simulink model "bldcControl"  (R2021b)
settings: Solver=VariableStepAuto  StartTime=0.0  StopTime=0.3  RelTol=1e-3
InitFcn:
  | modelData;
undefined symbols (not defined in the file or in its folder): inverter, motor
libraries: simulink x26, nesl_utility x13, fl_lib x7, ee_lib x6, simulink_extras x1
settings Model: Creator=andre  LastModifiedBy=andre
settings SolverCC: AlgebraicLoopSolver=TrustRegion
settings DebuggingCC: SFMachineParentedDataDiag=warning

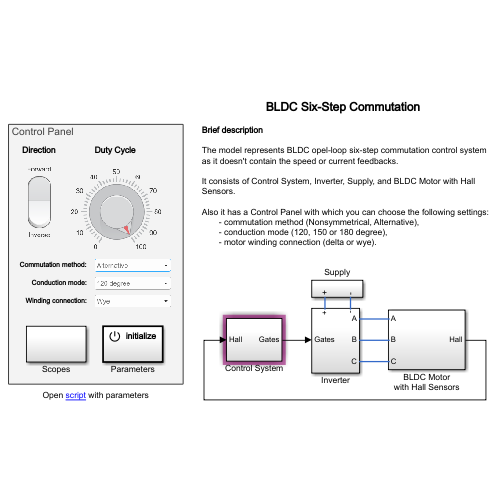
[thumbnail: Simulink's stored preview of the top-level diagram]
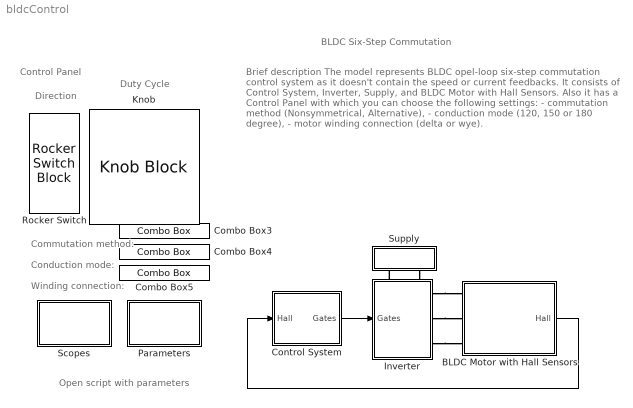
== system bldcControl ==
  note: Brief description
      |
      | The model represents BLDC opel-loop six-step commutation control system as it doesn't contain the speed or current feedbacks.
      |
      | It consists of Control System, Inverter, Supply, and BLDC Motor with Hall Sensors.
      |
      | Also it has a Control Panel with which you can choose the following settings: - commutation method (Nonsymmetrical, Alternative),
      | - conduction mode (120, 150 or 180 degree),
      | - motor winding connection (delta or wye).
  note: BLDC Six-Step Commutation
  note: Open script with parameters
  note: Direction
  note: Duty Cycle
  note: Commutation method:
  note: Control Panel
  note: Conduction mode:
  note: Winding connection:
  BLDC Motor with Hall Sensors : Subsystem
  Combo Box3 : ComboBox  LabelPosition=Hide  SelectedLabel=Alternative
      settings: Values={{'Nonsymmetrical (down)', 'Nonsymmetrical (up)', 'Alternative'}, [0 100 50]}
  Combo Box4 : ComboBox  LabelPosition=Hide  SelectedLabel=120 degree
      settings: Values={{'120 degree', '150 degree', '180 degree'}, [1 2 3]}
  Combo Box5 : ComboBox  LabelPosition=Hide  SelectedLabel=Wye
      settings: Values={{'Delta', 'Wye'}, [1 2]}
  Control System : Subsystem
  Inverter : Subsystem
      settings: PortSchema="{\"entries\":[{\"content\":{\"sides\":[{\"content\":{\"connectorIds\":[\"In1\"]},\"type\":\"ConnectorPlacement.EquallySpacedRectSide\",\"uuid\":\"39f629fa-0bd2-4f88-acf3-917ef1f8012c\"},{\"content\":{\"connectorIds\":[\"RConn1\",\"RConn2\",\"RConn3\"],\"side\":\"RIGHT\"},\"type\":\"ConnectorPlacement.EquallySpacedRectSide\",\"uuid\":\"8e31936c-1fbb-4376-88bf-295b0c5638c2\"},{\"content\":{\"connectorIds\":[\"LConn1\",\"LConn2\"],\"side\":\"TOP\"},\"type\":\"ConnectorPlacement.EquallySpacedRectSide\",\"uuid\":\"2e7c4c30-56fe-4abf-adf0-7801e76feedc\"},{\"content\":{\"connectorIds\":[],\"side\":\"BOTTOM\"},\"type\":\"ConnectorPlacement.EquallySpacedRectSide\",\"uuid\":\"fe44a21b-96bc-40f6-9ec6-e237835ad4c0\"},{\"content\":{\"connectorIds\":[],\"side\":\"HIDDEN\"},\"type\":\"ConnectorPlacement.EquallySpacedRectSide\",\"uuid\":\"0ee61edf-83e7-441c-a702-98ac80ee1211\"}]},\"type\":\"ConnectorPlacement.EquallySpacedConnector\",\"uuid\":\"7a564375-3113-4624-a173-7e6d668cb20c\"}],\"packageUris\":[\"http://schema.mathworks.com/mf0/Connector/R2020b\"],\"version\":\"1.0\"}"
  Knob : KnobBlock  LabelPosition=Hide  TickInterval=10
  Parameters : Subsystem  TreatAsAtomicUnit=on
  Rocker Switch : RockerSwitchBlock  LabelPosition=Hide
      settings: Values={{'Inverse', 'Forward'}, [1 0]}
  Scopes : Subsystem
  Supply : Subsystem
  wires:
  Control System/1(Gates) -> Inverter/1(Gates)
  BLDC Motor with Hall Sensors/1(Hall) -> Control System/1(Hall)
  connections:
  Inverter/RConn1 -- BLDC Motor with Hall Sensors/LConn1
  Supply/RConn2 -- Inverter/LConn2
  Inverter/RConn3 -- BLDC Motor with Hall Sensors/LConn3
  Inverter/RConn2 -- BLDC Motor with Hall Sensors/LConn2
  Inverter/LConn1 -- Supply/RConn1

== system bldcControl/BLDC Motor with Hall Sensors ==
  Hall Sensors : Subsystem
  Mechanical Rotational Reference1 : fl_lib/Mechanical/Rotational Elements/Mechanical Rotational Reference
  Motor : Subsystem  Variant=on
  A : PMIOPort  Side=Left
  B : PMIOPort  Port=2  Side=Left
  C : PMIOPort  Port=3  Side=Left
  Hall : Outport
  wires:
  Hall Sensors/1(Hall) -> Hall/1
  connections:
  Motor/LConn1 -- A/RConn1
  Motor/RConn1 -- Hall Sensors/LConn1
  Motor/LConn3 -- C/RConn1
  Motor/LConn2 -- B/RConn1
  Mechanical Rotational Reference1/LConn1 -- Motor/RConn2

== system bldcControl/Control System ==
  note: The control system is based on six-step commutation technique
      | which uses 120-degree, 150-degree, and 180-degree conduction modes.
      |
      | This control is described with the thuth table of 5 logical variables:
      | 1. DR (DiRection) is direction of the motor rotation
      | (0 - forward direction, 1 - inverse direction);
      | 2. H - Hall sensors signals;
      | 3. PR (PRoportion) determines the loading of switches
      | (PWM-based variable);
      | 4. SP (SPeed) is relative speed (PWM-based variable).
      |
      | When CM = 0, PR = 0 and lower switches are loaded more than
      | upper ones. When CM = 100, PR = 1 and upper switches are loaded
      | more than lower ones. When CM = 50, PR = 0.5, it means that
      | upper and lower switched are loaded uniformly during the commutation
      | interval.
      |
      | The commutation modes are called nonsymmentrical (down),
      | nonsymmentrical (up), and alternative, respectively.
  note: Description of commutation technique
  Hall : Inport
  CM : Constant  Value=50
  Direction : Constant  Value=0
  Duty Cycle : Constant  Value=100
  Logical variables formation : Subsystem
  Truth Tables : Subsystem  Variant=on
  Gates : Outport
  tag scope: Gates=global
  wires:
  Direction/1 -> Logical variables formation/1(DR)
  Hall/1 -> Logical variables formation/2(H)
  CM/1 -> Logical variables formation/3(PR)
  Duty Cycle/1 -> Logical variables formation/4(SP)
  Logical variables formation/1(LV) -> Truth Tables/1(LV)
  Truth Tables/1(Gates) -> Gates/1, [Gates]

== system bldcControl/Inverter ==
  Gates : Inport
  Converter (Three-Phase) : ee_lib/Semiconductors & Converters/Converters/Converter (Three-Phase)  port_option=ee.enum.threePhasePort.expanded  device_type=ee.enum.converters.switchingdevice.mosfet  Vf=0.8 V  Ron=4e-2 Ohm  Rds=inverter.Rds Ohm  Goff=inverter.Goffs 1/Ohm  Vgt=1 V  Vgt_off=-1 V  Ih=1 A  Vth=inverter.Uthr V  diode_param=ee.enum.converters.protectiondiode.nodynamics  diode_Vf=inverter.Udf V  diode_Ron=inverter.Ron Ohm  diode_Goff=inverter.Goff 1/Ohm  diode_C=50 nF  diode_iRM=-235 A  diode_iF=300 A  diode_idot=-50 A/us  diode_trr_param=ee.enum.converters.diodetrr.trr_factor  diode_trr_factor=3  diode_trr=15 us  diode_Qrr=1500 s*uA  snubber_type=ee.enum.converters.snubber.include  Cs=inverter.Csn F  Rs="inverter.Rsn  Ohm"
      settings: SourceProductBaseCode=PS  InternalSimscapePortConfiguration="{\"Bottom\":[],\"Left\":[{\"id\":\"G\",\"label\":\"G\",\"type\":\"foundation.electrical.twelve_phase\"},{\"id\":\"a\",\"label\":\"a\",\"type\":\"foundation.electrical.electrical\"},{\"id\":\"b\",\"label\":\"b\",\"type\":\"foundation.electrical.electrical\"},{\"id\":\"c\",\"label\":\"c\",\"type\":\"foundation.electrical.electrical\"}],\"Right\":[{\"id\":\"p\",\"label\":\"+\",\"type\":\"foundation.electrical.electrical\"},{\"id\":\"n\",\"label\":\"-\",\"type\":\"foundation.electrical.electrical\"}],\"Top\":[]}"
  Gate Driver : Subsystem
  Subsystem : Subsystem
      mask Display: disp('M')
  + : PMIOPort  Side=Left
  - : PMIOPort  Port=2  Side=Left
  A : PMIOPort  Port=3  Side=Right
  B : PMIOPort  Port=4  Side=Right
  C : PMIOPort  Port=5  Side=Right
  wires:
  Gates/1 -> Gate Driver/1(S)
  connections:
  Gate Driver/RConn1 -- Converter (Three-Phase)/LConn1
  Subsystem/RConn2 -- B/RConn1
  +/RConn1 -- Converter (Three-Phase)/RConn1
  Subsystem/LConn2 -- Converter (Three-Phase)/LConn3
  Subsystem/LConn3 -- Converter (Three-Phase)/LConn4
  Subsystem/LConn1 -- Converter (Three-Phase)/LConn2
  -/RConn1 -- Converter (Three-Phase)/RConn2
  Subsystem/RConn1 -- A/RConn1
  Subsystem/RConn3 -- C/RConn1

== system bldcControl/Parameters ==
  Control method : Constant
  Event Listener : EventListener  DisableCoverage=on  EventName=reset
  Terminator : Terminator
  Terminator1 : Terminator
  Wound type : Constant  Value=2
  wires:
  Control method/1 -> Terminator/1
  Wound type/1 -> Terminator1/1

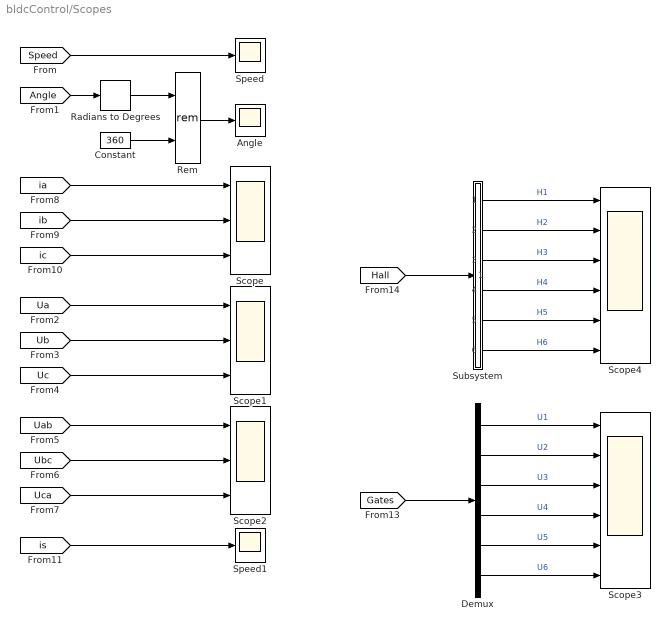
== system bldcControl/Scopes ==
  Angle : Scope
  Constant : Constant  Value=360
  Demux : Demux  Outputs=6
  Radians to Degrees : simulink_extras/Transformations/Radians to Degrees
  Rem : Math  Operator=rem  SaturateOnIntegerOverflow=on
  Scope : Scope  NumInputPorts=3
  Scope1 : Scope  NumInputPorts=3
  Scope2 : Scope  NumInputPorts=3
  Scope3 : Scope  NumInputPorts=6
  Scope4 : Scope  NumInputPorts=6
  Speed : Scope
  Speed1 : Scope
  Subsystem : Subsystem
  wires:
  [Angle] -> Radians to Degrees/1
  [ib] -> Scope/2
  [ia] -> Scope/1
  [ic] -> Scope/3
  [Ub] -> Scope1/2
  [Ua] -> Scope1/1
  [Uc] -> Scope1/3
  [Ubc] -> Scope2/2
  [Uab] -> Scope2/1
  [Uca] -> Scope2/3
  Rem/1 -> Angle/1
  Radians to Degrees/1 -> Rem/1
  Constant/1 -> Rem/2
  [is] -> Speed1/1
  [Speed] -> Speed/1
  [Gates] -> Demux/1
  [Hall] -> Subsystem/1(In1)
  Demux/1 -> Scope3/1  "U1"
  Demux/2 -> Scope3/2  "U2"
  Demux/3 -> Scope3/3  "U3"
  Demux/4 -> Scope3/4  "U4"
  Demux/5 -> Scope3/5  "U5"
  Demux/6 -> Scope3/6  "U6"
  Subsystem/1(H1) -> Scope4/1  "H1"
  Subsystem/2(H2) -> Scope4/2  "H2"
  Subsystem/3(H3) -> Scope4/3  "H3"
  Subsystem/4(H4) -> Scope4/4  "H4"
  Subsystem/5(H5) -> Scope4/5  "H5"
  Subsystem/6(H6) -> Scope4/6  "H6"

== system bldcControl/Supply ==
  DC Voltage Source : fl_lib/Electrical/Electrical Sources/DC Voltage Source  v0=motor.Us V
  Electrical Reference2 : fl_lib/Electrical/Electrical Elements/Electrical Reference
  Solver Configuration : nesl_utility/Solver Configuration  PhysicalDomain=network_engine_domain  SubClassName=solver  LeftPortType=input  RightPortType=generic  Tones=[]  Harmonics=[]  SimulateNoise=off  Profile=off  UseLocalSampling=off  EnableSwitchedLinearOptims=on  FrequencyDomain=off  UseCCode=off  RelTol=0.001  AbsTol=1e-06  MinStep=1e-09  ToWorkspace=off  RevertToSquareIcSolve=off  NumHomotopyIterations=100  PhasorMode=off  PhasorModeNumHarmonics=1  DoDC=off  ResidualTolerance=1e-09  UseLocalSolver=on  LocalSolverChoice=NE_BACKWARD_EULER_ADVANCER  LocalSolverSampleTime=Ts  DoFixedCost=on  MaxNonlinIter=4  MaxModeIter=2  ComputeImpulses=off  ImpulseIterations=2  LinearAlgebra=auto  EquationFormulation=NE_TIME_EF  DelaysMemoryBudget=1024  AutomaticFiltering=off  FilteringTimeConstant=0.001  PartitionStorageMethod=AS_NEEDED  PartitionMemoryBudget=1024  PartitionMethod=ROBUST
      settings: SourceProductBaseCode=PW,SS
  Subsystem : Subsystem
      mask Display: disp('A')
  + : PMIOPort  Side=Right
  - : PMIOPort  Port=2  Side=Right
  connections:
  DC Voltage Source/RConn1 -- Electrical Reference2/LConn1 -- Solver Configuration/RConn1 -- -/RConn1
  Subsystem/RConn1 -- +/RConn1
  Subsystem/LConn1 -- DC Voltage Source/LConn1

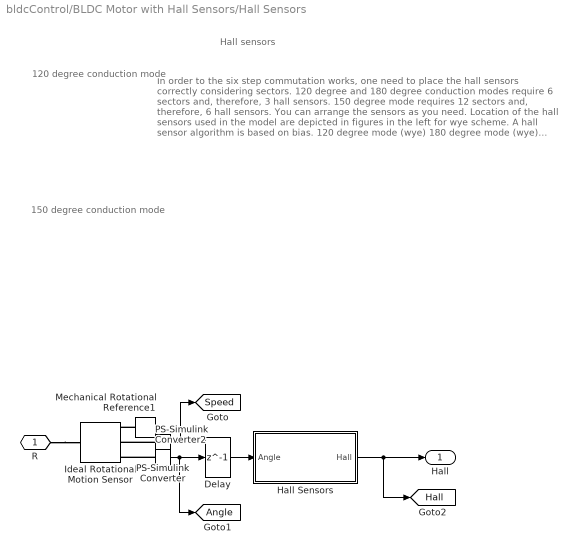
== system bldcControl/BLDC Motor with Hall Sensors/Hall Sensors ==
  note: In order to the six step commutation works, one need to place the hall sensors correctly considering sectors.
      |
      | 120 degree and 180 degree conduction modes require 6 sectors and, therefore, 3 hall sensors. 150 degree mode requires 12 sectors and, therefore, 6 hall sensors.
      |
      | You can arrange the sensors as you need. Location of the hall sensors used in the model are depicted in figures in the left for wye scheme.
      |
      | A hall sensor algorithm is based on bias.
      |
      | 120 degree mode (wye)    180 degree mode (wye)    150 degree mode (wye)
      | 	H   | Bias				H   | Bias				H   | Bias
      | 	H1 | 0					H1 | -pi/6				H1 | pi/3
      | 	H2 | 2*pi/3				H2 | pi/2					H2 | pi/6
      | 	H3 | -2*pi/3				H3 | -5*pi/6				H3 | 0
      | 													H4 | -pi/6
      | 													H5 | -pi/3
      | 													H6 | -pi/2
      |
      | For delta scheme, all corresponding hall sensors are moved clockwise
      | by 30 degrees relative to wye scheme.
  note: 120 degree
      | conduction mode
  note: Hall sensors
  note: 150 degree
      | conduction mode
  Delay : Delay  DelayLength=1
  Hall Sensors : Subsystem  Variant=on
  Ideal Rotational Motion Sensor : fl_lib/Mechanical/Mechanical Sensors/Ideal Rotational Motion Sensor  wrap_angle=simscape.enum.onoff.off  offset=0 deg
  Mechanical Rotational Reference1 : fl_lib/Mechanical/Rotational Elements/Mechanical Rotational Reference
  PS-Simulink Converter : nesl_utility/PS-Simulink Converter  PhysicalDomain=network_engine_domain  SubClassName=ps_output  LeftPortType=input  RightPortType=output  PseudoPeriodic=off  Frequencies=[]  Unit=rpm  AffineConversion=off
      settings: SourceProductBaseCode=PW,SS
  PS-Simulink Converter2 : nesl_utility/PS-Simulink Converter  PhysicalDomain=network_engine_domain  SubClassName=ps_output  LeftPortType=input  RightPortType=output  PseudoPeriodic=off  Frequencies=[]  Unit=rad  AffineConversion=off
      settings: SourceProductBaseCode=PW,SS
  R : PMIOPort  Side=Left
  Hall : Outport
  tag scope: Angle=global, Hall=global, Speed=global
  wires:
  Delay/1 -> Hall Sensors/1(Angle)
  PS-Simulink Converter2/1 -> [Angle], Delay/1
  Hall Sensors/1(Hall) -> [Hall], Hall/1
  PS-Simulink Converter/1 -> [Speed]
  connections:
  PS-Simulink Converter2/LConn1 -- Ideal Rotational Motion Sensor/RConn3
  PS-Simulink Converter/LConn1 -- Ideal Rotational Motion Sensor/RConn2
  Mechanical Rotational Reference1/LConn1 -- Ideal Rotational Motion Sensor/RConn1
  R/RConn1 -- Ideal Rotational Motion Sensor/LConn1

== system bldcControl/BLDC Motor with Hall Sensors/Motor ==
  Delta : Subsystem  VariantControl=DELTA_WOUND
  Wye : Subsystem  VariantControl=WYE_WOUND
  A : PMIOPort  Side=Left
  B : PMIOPort  Port=2  Side=Left
  C : PMIOPort  Port=3  Side=Left
  R : PMIOPort  Port=4  Side=Right
  Сase : PMIOPort  Port=5  Side=Right

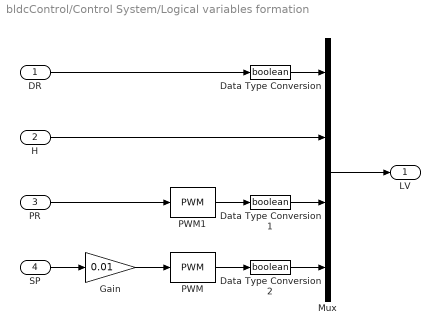
== system bldcControl/Control System/Logical variables formation ==
  DR : Inport
  H : Inport  Port=2
  PR : Inport  Port=3
  SP : Inport  Port=4
  Data Type Conversion : DataTypeConversion  OutDataTypeStr=boolean
  Data Type Conversion1 : DataTypeConversion  OutDataTypeStr=boolean
  Data Type Conversion2 : DataTypeConversion  OutDataTypeStr=boolean
  Gain : Gain  Gain=0.01
  Mux : Mux
  PWM : simulink/Discontinuities/PWM  DisableCoverage=on  Period=1/inverter.f  DisallowZeroDutyCycle=off  RunAtFixedTimeIntervals=off  SampleTime=0.1
  PWM1 : simulink/Discontinuities/PWM  DisableCoverage=on  Period=2/inverter.f  DisallowZeroDutyCycle=off  RunAtFixedTimeIntervals=off  SampleTime=0.1
  LV : Outport
  wires:
  Data Type Conversion/1 -> Mux/1
  DR/1 -> Data Type Conversion/1
  SP/1 -> Gain/1
  PR/1 -> PWM1/1
  PWM1/1 -> Data Type Conversion1/1
  Gain/1 -> PWM/1
  PWM/1 -> Data Type Conversion2/1
  Data Type Conversion1/1 -> Mux/3
  Mux/1 -> LV/1
  Data Type Conversion2/1 -> Mux/4
  H/1 -> Mux/2

== system bldcControl/Control System/Truth Tables ==
  LV : Inport
  120 degree : Subsystem  VariantControl=DEG120
  150 degree : Subsystem  VariantControl=DEG150
  180 degree : Subsystem  VariantControl=DEG180
  Gates : Outport

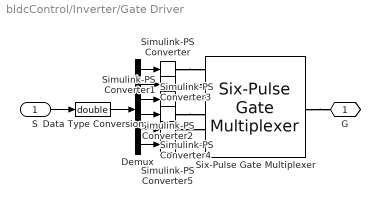
== system bldcControl/Inverter/Gate Driver ==
  S : Inport
  Data Type Conversion : DataTypeConversion  OutDataTypeStr=double
  Demux : Demux  Outputs=6
  Simulink-PS Converter{,1..5} (6 alike) : nesl_utility/Simulink-PS Converter  PhysicalDomain=network_engine_domain  SubClassName=ps_input  LeftPortType=input  RightPortType=output  PseudoPeriodic=off  Frequencies=[]  NoiseDistribution=none  NoiseParameters=[]  Unit=1  AffineConversion=off  FilteringAndDerivatives=provide  SimscapeFilterOrder=1  InputFilterTimeConstant=0.001  UdotUserProvided=0
      settings: SourceProductBaseCode=PW,SS
  Six-Pulse Gate Multiplexer : ee_lib/Semiconductors & Converters/Converters/Six-Pulse Gate Multiplexer  port_option=ee.enum.controlport.ps
      settings: SourceProductBaseCode=PS
  G : PMIOPort  Side=Right
  wires:
  Demux/3 -> Simulink-PS Converter2/1
  Demux/2 -> Simulink-PS Converter1/1
  Demux/6 -> Simulink-PS Converter5/1
  Demux/5 -> Simulink-PS Converter4/1
  Demux/4 -> Simulink-PS Converter3/1
  Demux/1 -> Simulink-PS Converter/1
  Data Type Conversion/1 -> Demux/1
  S/1 -> Data Type Conversion/1
  connections:
  Simulink-PS Converter4/RConn1 -- Six-Pulse Gate Multiplexer/LConn5
  Six-Pulse Gate Multiplexer/LConn6 -- Simulink-PS Converter5/RConn1
  Simulink-PS Converter3/RConn1 -- Six-Pulse Gate Multiplexer/LConn4
  Simulink-PS Converter1/RConn1 -- Six-Pulse Gate Multiplexer/LConn2
  Six-Pulse Gate Multiplexer/LConn3 -- Simulink-PS Converter2/RConn1
  Simulink-PS Converter/RConn1 -- Six-Pulse Gate Multiplexer/LConn1
  Six-Pulse Gate Multiplexer/RConn1 -- G/RConn1

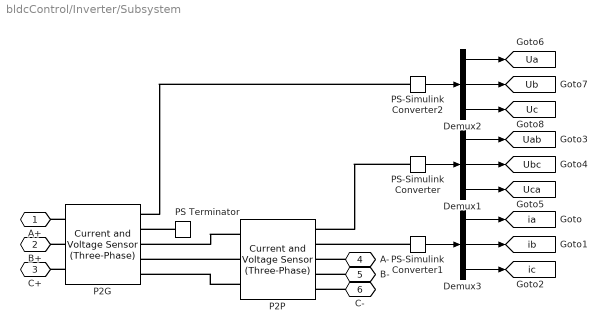
== system bldcControl/Inverter/Subsystem ==
  Demux1 : Demux  Outputs=3
  Demux2 : Demux  Outputs=3
  Demux3 : Demux  Outputs=3
  P2G : ee_lib/Sensors & Transducers/Current and Voltage Sensor (Three-Phase)  vMeasurementType=ee.enum.vmeasurement.lg  outputUnit=ee.enum.unit.si  SRated=100e6 V*A  VRated=24e3 V  I_specify=off  I_priority=None  I=[ 0 0 0 ] A  I_nominal_specify=off  I_nominal_unit=A  I_nominal_value=1  V_specify=off  V_priority=None  V=[ 0 0 0 ] V  V_nominal_specify=off  V_nominal_unit=V  V_nominal_value=1
      settings: SourceProductBaseCode=PS  InternalSimscapePortConfiguration="{\"Bottom\":[],\"Left\":[{\"id\":\"a1\",\"label\":\"a1\",\"type\":\"foundation.electrical.electrical\"},{\"id\":\"b1\",\"label\":\"b1\",\"type\":\"foundation.electrical.electrical\"},{\"id\":\"c1\",\"label\":\"c1\",\"type\":\"foundation.electrical.electrical\"}],\"Right\":[{\"id\":\"V_output\",\"label\":\"V\",\"type\":\"output\"},{\"id\":\"I_output\",\"label\":\"I\",\"type\":\"output\"},{\"id\":\"a2\",\"label\":\"a2\",\"type\":\"foundation.electrical.electrical\"},{\"id\":\"b2\",\"label\":\"b2\",\"type\":\"foundation.electrical.electrical\"},{\"id\":\"c2\",\"label\":\"c2\",\"type\":\"foundation.electrical.electrical\"}],\"Top\":[]}"
  P2P : ee_lib/Sensors & Transducers/Current and Voltage Sensor (Three-Phase)  vMeasurementType=ee.enum.vmeasurement.ll  outputUnit=ee.enum.unit.si  SRated=100e6 V*A  VRated=24e3 V  I_specify=off  I_priority=None  I=[ 0 0 0 ] A  I_nominal_specify=off  I_nominal_unit=A  I_nominal_value=1  V_specify=off  V_priority=None  V=[ 0 0 0 ] V  V_nominal_specify=off  V_nominal_unit=V  V_nominal_value=1
      settings: SourceProductBaseCode=PS  InternalSimscapePortConfiguration="{\"Bottom\":[],\"Left\":[{\"id\":\"a1\",\"label\":\"a1\",\"type\":\"foundation.electrical.electrical\"},{\"id\":\"b1\",\"label\":\"b1\",\"type\":\"foundation.electrical.electrical\"},{\"id\":\"c1\",\"label\":\"c1\",\"type\":\"foundation.electrical.electrical\"}],\"Right\":[{\"id\":\"V_output\",\"label\":\"V\",\"type\":\"output\"},{\"id\":\"I_output\",\"label\":\"I\",\"type\":\"output\"},{\"id\":\"a2\",\"label\":\"a2\",\"type\":\"foundation.electrical.electrical\"},{\"id\":\"b2\",\"label\":\"b2\",\"type\":\"foundation.electrical.electrical\"},{\"id\":\"c2\",\"label\":\"c2\",\"type\":\"foundation.electrical.electrical\"}],\"Top\":[]}"
  PS Terminator : fl_lib/Physical Signals/Sinks/PS Terminator
  PS-Simulink Converter : nesl_utility/PS-Simulink Converter  PhysicalDomain=network_engine_domain  SubClassName=ps_output  LeftPortType=input  RightPortType=output  PseudoPeriodic=off  Frequencies=[]  Unit=inherit  AffineConversion=off
      settings: SourceProductBaseCode=PW,SS
  PS-Simulink Converter1 : nesl_utility/PS-Simulink Converter  PhysicalDomain=network_engine_domain  SubClassName=ps_output  LeftPortType=input  RightPortType=output  PseudoPeriodic=off  Frequencies=[]  Unit=inherit  AffineConversion=off
      settings: SourceProductBaseCode=PW,SS
  PS-Simulink Converter2 : nesl_utility/PS-Simulink Converter  PhysicalDomain=network_engine_domain  SubClassName=ps_output  LeftPortType=input  RightPortType=output  PseudoPeriodic=off  Frequencies=[]  Unit=inherit  AffineConversion=off
      settings: SourceProductBaseCode=PW,SS
  A+ : PMIOPort  Side=Left
  B+ : PMIOPort  Port=2  Side=Left
  C+ : PMIOPort  Port=3  Side=Left
  A- : PMIOPort  Port=4  Side=Right
  B- : PMIOPort  Port=5  Side=Right
  C- : PMIOPort  Port=6  Side=Right
  tag scope: Ua=global, Uab=global, Ub=global, Ubc=global, Uc=global, Uca=global, ia=global, ib=global, ic=global
  wires:
  PS-Simulink Converter1/1 -> Demux3/1
  PS-Simulink Converter/1 -> Demux1/1
  PS-Simulink Converter2/1 -> Demux2/1
  Demux3/1 -> [ia]
  Demux3/2 -> [ib]
  Demux3/3 -> [ic]
  Demux1/1 -> [Uab]
  Demux1/2 -> [Ubc]
  Demux1/3 -> [Uca]
  Demux2/1 -> [Ua]
  Demux2/2 -> [Ub]
  Demux2/3 -> [Uc]
  connections:
  P2G/LConn1 -- A+/RConn1
  P2G/LConn2 -- B+/RConn1
  P2G/LConn3 -- C+/RConn1
  PS Terminator/LConn1 -- P2G/RConn2
  A-/RConn1 -- P2P/RConn3
  B-/RConn1 -- P2P/RConn4
  C-/RConn1 -- P2P/RConn5
  PS-Simulink Converter1/LConn1 -- P2P/RConn2
  PS-Simulink Converter/LConn1 -- P2P/RConn1
  PS-Simulink Converter2/LConn1 -- P2G/RConn1
  P2P/LConn1 -- P2G/RConn3
  P2P/LConn2 -- P2G/RConn4
  P2P/LConn3 -- P2G/RConn5

== system bldcControl/Scopes/Subsystem ==
  In1 : Inport
  Demux : Demux  Outputs=6
  Variant Subsystem : Subsystem  Variant=on
  H1 : Outport
  H2 : Outport  Port=2
  H3 : Outport  Port=3
  H4 : Outport  Port=4
  H5 : Outport  Port=5
  H6 : Outport  Port=6
  wires:
  In1/1 -> Variant Subsystem/1(In1)
  Variant Subsystem/1(Out1) -> Demux/1
  Demux/5 -> H5/1
  Demux/6 -> H6/1
  Demux/1 -> H1/1
  Demux/2 -> H2/1
  Demux/3 -> H3/1
  Demux/4 -> H4/1

== system bldcControl/Supply/Subsystem ==
  Current Sensor : fl_lib/Electrical/Electrical Sensors/Current Sensor
  PS-Simulink Converter : nesl_utility/PS-Simulink Converter  PhysicalDomain=network_engine_domain  SubClassName=ps_output  LeftPortType=input  RightPortType=output  PseudoPeriodic=off  Frequencies=[]  Unit=inherit  AffineConversion=off
      settings: SourceProductBaseCode=PW,SS
  + : PMIOPort  Side=Left
  - : PMIOPort  Port=2  Side=Right
  tag scope: is=global
  wires:
  PS-Simulink Converter/1 -> [is]
  connections:
  +/RConn1 -- Current Sensor/LConn1
  Current Sensor/RConn2 -- -/RConn1
  PS-Simulink Converter/LConn1 -- Current Sensor/RConn1

== system bldcControl/BLDC Motor with Hall Sensors/Hall Sensors/Hall Sensors ==
  Angle : Inport
  Delta : Subsystem  VariantControl=DELTA_WOUND
  Wye : Subsystem  VariantControl=WYE_WOUND
  Hall : Outport

== system bldcControl/BLDC Motor with Hall Sensors/Motor/Delta ==
  BLDC : ee_lib/Electromechanical/Permanent Magnet/BLDC  port_option=ee.enum.threePhasePort.expanded  winding_type=ee.enum.statorconnection.delta  rotor_param=ee.enum.pmsm.backemf.trapezoidflux  pm_flux_linkage=(2/3)*(motor.Cm/motor.p) Wb  theta_constant=pi / (2*motor.p) rad  emf_max=2.71 V  w_meas=1000 rpm  DphiDtheta_tab=[0, -.1528, -.1528, .1528, .1528, 0] Wb/rad  back_emf_tab=[0, -9.6, -9.6, 9.6, 9.6, 0] V  rotor_angle_tab=[0, 7.5, 22.5, 37.5, 52.5, 60] deg  nPolePairs=motor.p  axes_param=ee.enum.rotorangle.daxis  stator_param=ee.enum.statorparam.LsLmMs  machine_param=ee.enum.dqparameterization.constant  Ld=0.00022 H  Lq=0.00022 H  idVec=[-200, 0, 200] A  iqVec=[-200, 0, 200] A  LdMatrix=0.00022 * ones(3, 3) H  LqMatrix=0.00022 * ones(3, 3) H  L0=0.00016 H  Ls=motor.L H  Lm=0 H  Ms=0 H  Rs=motor.R Ohm  zero_sequence=ee.enum.park.zerosequence.exclude  loss_param=ee.enum.ironloss.none  losses_oc=[0, 0, 0] W  losses_sc=[0, 0, 0] W  f_losses=60 Hz  Isc_losses=95 A  J=motor.J kg*m^2  lam=motor.Bm N*m/(rad/s)  i_d_specify=off  i_d_priority=None  i_d=0 A  i_d_nominal_specify=off  i_d_nominal_unit=A  i_d_nominal_value=1  i_q_specify=off  i_q_priority=None  i_q=0 A  i_q_nominal_specify=off  i_q_nominal_unit=A  i_q_nominal_value=1  torque_specify=off  torque_priority=None  torque=0 N*m  torque_nominal_specify=off  torque_nominal_unit=N*m  torque_nominal_value=1  angular_velocity_specify=off  angular_velocity_priority=High  angular_velocity=0 rpm  angular_velocity_nominal_specify=off  angular_velocity_nominal_unit=rpm  angular_velocity_nominal_value=1  angular_position_specify=off  angular_position_priority=High  angular_position=0 deg  angular_position_nominal_specify=off  angular_position_nominal_unit=deg  angular_position_nominal_value=1  alpha=3.93e-3 1/K  alpha_flux=-0.001 1/K  Tmeas=298.15 K  stator_thermal_mass=100 J/K  rotor_thermal_mass=200 J/K  Rm_percent_rotor=90  Rd_percent_rotor=30  temperatureA_specify=off  temperatureA_priority=High  temperatureA=25 degC  temperatureA_nominal_specify=off  temperatureA_nominal_unit=degC  temperatureA_nominal_value=1  temperatureB_specify=off  temperatureB_priority=High  temperatureB=25 degC  temperatureB_nominal_specify=off  temperatureB_nominal_unit=degC  temperatureB_nominal_value=1  temperatureC_specify=off  temperatureC_priority=High  temperatureC=25 degC  temperatureC_nominal_specify=off  temperatureC_nominal_unit=degC  temperatureC_nominal_value=1  temperatureR_specify=off  temperatureR_priority=High  temperatureR=25 degC  temperatureR_nominal_specify=off  temperatureR_nominal_unit=degC  temperatureR_nominal_value=1
      settings: SourceProductBaseCode=PS  InternalSimscapePortConfiguration="{\"Bottom\":[],\"Left\":[{\"id\":\"a\",\"label\":\"a\",\"type\":\"foundation.electrical.electrical\"},{\"id\":\"b\",\"label\":\"b\",\"type\":\"foundation.electrical.electrical\"},{\"id\":\"c\",\"label\":\"c\",\"type\":\"foundation.electrical.electrical\"}],\"Right\":[{\"id\":\"R\",\"label\":\"R\",\"type\":\"foundation.mechanical.rotational.rotational\"},{\"id\":\"C\",\"label\":\"C\",\"type\":\"foundation.mechanical.rotational.rotational\"}],\"Top\":[]}"
  A : PMIOPort  Side=Left
  B : PMIOPort  Port=2  Side=Left
  C : PMIOPort  Port=3  Side=Left
  R : PMIOPort  Port=4  Side=Right
  Сase : PMIOPort  Port=5  Side=Right
  connections:
  C/RConn1 -- BLDC/LConn3
  B/RConn1 -- BLDC/LConn2
  A/RConn1 -- BLDC/LConn1
  R/RConn1 -- BLDC/RConn1
  Сase/RConn1 -- BLDC/RConn2

== system bldcControl/BLDC Motor with Hall Sensors/Motor/Wye ==
  BLDC : ee_lib/Electromechanical/Permanent Magnet/BLDC  port_option=ee.enum.threePhasePort.expanded  winding_type=ee.enum.statorconnection.wye  rotor_param=ee.enum.pmsm.backemf.trapezoidflux  pm_flux_linkage=(2/3)*(motor.Cm/motor.p) Wb  theta_constant=pi / (2*motor.p) rad  emf_max=2.71 V  w_meas=1000 rpm  DphiDtheta_tab=[0, -.1528, -.1528, .1528, .1528, 0] Wb/rad  back_emf_tab=[0, -9.6, -9.6, 9.6, 9.6, 0] V  rotor_angle_tab=[0, 7.5, 22.5, 37.5, 52.5, 60] deg  nPolePairs=motor.p  axes_param=ee.enum.rotorangle.daxis  stator_param=ee.enum.statorparam.LsLmMs  machine_param=ee.enum.dqparameterization.constant  Ld=0.00022 H  Lq=0.00022 H  idVec=[-200, 0, 200] A  iqVec=[-200, 0, 200] A  LdMatrix=0.00022 * ones(3, 3) H  LqMatrix=0.00022 * ones(3, 3) H  L0=0.00016 H  Ls=motor.L H  Lm=0 H  Ms=0 H  Rs=motor.R Ohm  zero_sequence=ee.enum.park.zerosequence.exclude  loss_param=ee.enum.ironloss.none  losses_oc=[0, 0, 0] W  losses_sc=[0, 0, 0] W  f_losses=60 Hz  Isc_losses=95 A  J=motor.J kg*m^2  lam=motor.Bm N*m/(rad/s)  i_d_specify=off  i_d_priority=None  i_d=0 A  i_d_nominal_specify=off  i_d_nominal_unit=A  i_d_nominal_value=1  i_q_specify=off  i_q_priority=None  i_q=0 A  i_q_nominal_specify=off  i_q_nominal_unit=A  i_q_nominal_value=1  torque_specify=off  torque_priority=None  torque=0 N*m  torque_nominal_specify=off  torque_nominal_unit=N*m  torque_nominal_value=1  angular_velocity_specify=off  angular_velocity_priority=High  angular_velocity=0 rpm  angular_velocity_nominal_specify=off  angular_velocity_nominal_unit=rpm  angular_velocity_nominal_value=1  angular_position_specify=off  angular_position_priority=High  angular_position=180 deg  angular_position_nominal_specify=off  angular_position_nominal_unit=deg  angular_position_nominal_value=1  alpha=3.93e-3 1/K  alpha_flux=-0.001 1/K  Tmeas=298.15 K  stator_thermal_mass=100 J/K  rotor_thermal_mass=200 J/K  Rm_percent_rotor=90  Rd_percent_rotor=30  temperatureA_specify=off  temperatureA_priority=High  temperatureA=25 degC  temperatureA_nominal_specify=off  temperatureA_nominal_unit=degC  temperatureA_nominal_value=1  temperatureB_specify=off  temperatureB_priority=High  temperatureB=25 degC  temperatureB_nominal_specify=off  temperatureB_nominal_unit=degC  temperatureB_nominal_value=1  temperatureC_specify=off  temperatureC_priority=High  temperatureC=25 degC  temperatureC_nominal_specify=off  temperatureC_nominal_unit=degC  temperatureC_nominal_value=1  temperatureR_specify=off  temperatureR_priority=High  temperatureR=25 degC  temperatureR_nominal_specify=off  temperatureR_nominal_unit=degC  temperatureR_nominal_value=1
      settings: SourceProductBaseCode=PS  InternalSimscapePortConfiguration="{\"Bottom\":[],\"Left\":[{\"id\":\"a\",\"label\":\"a\",\"type\":\"foundation.electrical.electrical\"},{\"id\":\"b\",\"label\":\"b\",\"type\":\"foundation.electrical.electrical\"},{\"id\":\"c\",\"label\":\"c\",\"type\":\"foundation.electrical.electrical\"}],\"Right\":[{\"id\":\"R\",\"label\":\"R\",\"type\":\"foundation.mechanical.rotational.rotational\"},{\"id\":\"C\",\"label\":\"C\",\"type\":\"foundation.mechanical.rotational.rotational\"}],\"Top\":[]}"
  A : PMIOPort  Side=Left
  B : PMIOPort  Port=2  Side=Left
  C : PMIOPort  Port=3  Side=Left
  R : PMIOPort  Port=4  Side=Right
  Сase : PMIOPort  Port=5  Side=Right
  connections:
  C/RConn1 -- BLDC/LConn3
  B/RConn1 -- BLDC/LConn2
  A/RConn1 -- BLDC/LConn1
  R/RConn1 -- BLDC/RConn1
  Сase/RConn1 -- BLDC/RConn2

== system bldcControl/Control System/Truth Tables/120 degree ==
  LV : Inport
  120deg : CombinatorialLogic  TruthTable=truthTable120d
  Gates : Outport
  wires:
  120deg/1 -> Gates/1
  LV/1 -> 120deg/1

== system bldcControl/Control System/Truth Tables/150 degree ==
  LV : Inport
  120deg : CombinatorialLogic  TruthTable=truthTable150d
  Gates : Outport
  wires:
  120deg/1 -> Gates/1
  LV/1 -> 120deg/1

== system bldcControl/Control System/Truth Tables/180 degree ==
  LV : Inport
  120deg : CombinatorialLogic  TruthTable=truthTable180d
  Gates : Outport
  wires:
  120deg/1 -> Gates/1
  LV/1 -> 120deg/1

== system bldcControl/Scopes/Subsystem/Variant Subsystem ==
  In1 : Inport
  120/180 degree : Subsystem  VariantControl=DEG120_180
  150 degree : Subsystem  VariantControl=DEG150
  Out1 : Outport

== system bldcControl/BLDC Motor with Hall Sensors/Hall Sensors/Hall Sensors/Delta ==
  Angle : Inport
  Variant Subsystem : Subsystem  Variant=on
  Hall : Outport
  wires:
  Variant Subsystem/1(Hall) -> Hall/1
  Angle/1 -> Variant Subsystem/1(Angle)

== system bldcControl/BLDC Motor with Hall Sensors/Hall Sensors/Hall Sensors/Wye ==
  Angle : Inport
  Variant Subsystem : Subsystem  Variant=on
  Hall : Outport
  wires:
  Variant Subsystem/1(Hall) -> Hall/1
  Angle/1 -> Variant Subsystem/1(Angle)

== system bldcControl/Scopes/Subsystem/Variant Subsystem/120//180 degree ==
  In1 : Inport
  Demux : Demux  Outputs=3
  Ground : Ground
  Mux : Mux  Inputs=6
  Out1 : Outport
  wires:
  Mux/1 -> Out1/1
  Demux/3 -> Mux/3
  Demux/2 -> Mux/2
  Demux/1 -> Mux/1
  In1/1 -> Demux/1
  Ground/1 -> Mux/6, Mux/4, Mux/5

== system bldcControl/Scopes/Subsystem/Variant Subsystem/150 degree ==
  In1 : Inport
  Out1 : Outport
  wires:
  In1/1 -> Out1/1

== system bldcControl/BLDC Motor with Hall Sensors/Hall Sensors/Hall Sensors/Delta/Variant Subsystem ==
  Angle : Inport
  120 degree : Subsystem  VariantControl=DEG120
  150 degree : Subsystem  VariantControl=DEG150
  180 degree : Subsystem  VariantControl=DEG180
  Hall : Outport

== system bldcControl/BLDC Motor with Hall Sensors/Hall Sensors/Hall Sensors/Wye/Variant Subsystem ==
  Angle : Inport
  120 degree : Subsystem  VariantControl=DEG120
  150 degree : Subsystem  VariantControl=DEG150
  180 degree : Subsystem  VariantControl=DEG180
  Hall : Outport

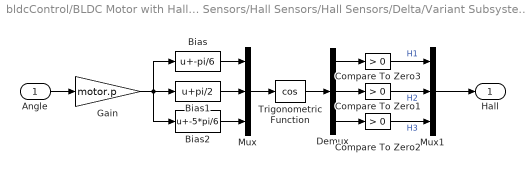
== system bldcControl/BLDC Motor with Hall Sensors/Hall Sensors/Hall Sensors/Delta/Variant Subsystem/120 degree ==
  Angle : Inport
  Bias : Bias  Bias=-pi/6
  Bias1 : Bias  Bias=pi/2
  Bias2 : Bias  Bias=-5*pi/6
  Compare To Zero1 : simulink/Logic and Bit Operations/Compare To Zero  relop=>  OutDataTypeStr=boolean
  Compare To Zero2 : simulink/Logic and Bit Operations/Compare To Zero  relop=>  OutDataTypeStr=boolean
  Compare To Zero3 : simulink/Logic and Bit Operations/Compare To Zero  relop=>  OutDataTypeStr=boolean
  Demux : Demux  Outputs=3
  Gain : Gain  Gain=motor.p
  Mux : Mux  Inputs=3
  Mux1 : Mux  Inputs=3
  Trigonometric Function : Trigonometry  Operator=cos
  Hall : Outport
  wires:
  Bias2/1 -> Mux/3
  Mux1/1 -> Hall/1
  Demux/3 -> Compare To Zero2/1
  Mux/1 -> Trigonometric Function/1
  Gain/1 -> Bias2/1, Bias1/1, Bias/1
  Compare To Zero1/1 -> Mux1/2  "H2"
  Compare To Zero3/1 -> Mux1/1  "H1"
  Trigonometric Function/1 -> Demux/1
  Bias1/1 -> Mux/2
  Bias/1 -> Mux/1
  Compare To Zero2/1 -> Mux1/3  "H3"
  Demux/2 -> Compare To Zero1/1
  Angle/1 -> Gain/1
  Demux/1 -> Compare To Zero3/1

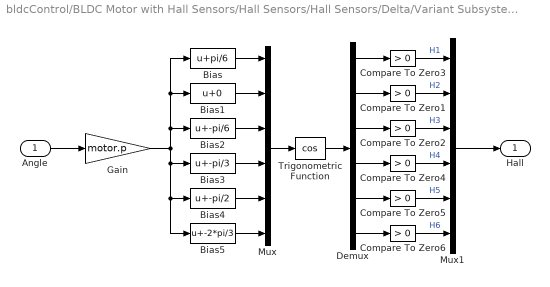
== system bldcControl/BLDC Motor with Hall Sensors/Hall Sensors/Hall Sensors/Delta/Variant Subsystem/150 degree ==
  Angle : Inport
  Bias : Bias  Bias=pi/6
  Bias1 : Bias
  Bias2 : Bias  Bias=-pi/6
  Bias3 : Bias  Bias=-pi/3
  Bias4 : Bias  Bias=-pi/2
  Bias5 : Bias  Bias=-2*pi/3
  Compare To Zero{1..6} (6 alike) : simulink/Logic and Bit Operations/Compare To Zero  relop=>  OutDataTypeStr=boolean
  Demux : Demux  Outputs=6
  Gain : Gain  Gain=motor.p
  Mux : Mux  Inputs=6
  Mux1 : Mux  Inputs=6
  Trigonometric Function : Trigonometry  Operator=cos
  Hall : Outport
  wires:
  Bias5/1 -> Mux/6
  Compare To Zero6/1 -> Mux1/6  "H6"
  Bias4/1 -> Mux/5
  Bias3/1 -> Mux/4
  Mux1/1 -> Hall/1
  Bias2/1 -> Mux/3
  Bias1/1 -> Mux/2
  Demux/1 -> Compare To Zero3/1
  Compare To Zero4/1 -> Mux1/4  "H4"
  Demux/6 -> Compare To Zero6/1
  Bias/1 -> Mux/1
  Demux/5 -> Compare To Zero5/1
  Mux/1 -> Trigonometric Function/1
  Compare To Zero5/1 -> Mux1/5  "H5"
  Demux/4 -> Compare To Zero4/1
  Compare To Zero3/1 -> Mux1/1  "H1"
  Angle/1 -> Gain/1
  Trigonometric Function/1 -> Demux/1
  Demux/2 -> Compare To Zero1/1
  Gain/1 -> Bias2/1, Bias1/1, Bias/1, Bias3/1, Bias4/1, Bias5/1
  Demux/3 -> Compare To Zero2/1
  Compare To Zero1/1 -> Mux1/2  "H2"
  Compare To Zero2/1 -> Mux1/3  "H3"

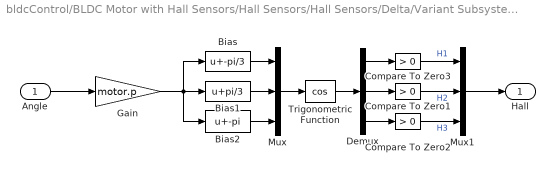
== system bldcControl/BLDC Motor with Hall Sensors/Hall Sensors/Hall Sensors/Delta/Variant Subsystem/180 degree ==
  Angle : Inport
  Bias : Bias  Bias=-pi/3
  Bias1 : Bias  Bias=pi/3
  Bias2 : Bias  Bias=-pi
  Compare To Zero1 : simulink/Logic and Bit Operations/Compare To Zero  relop=>  OutDataTypeStr=boolean
  Compare To Zero2 : simulink/Logic and Bit Operations/Compare To Zero  relop=>  OutDataTypeStr=boolean
  Compare To Zero3 : simulink/Logic and Bit Operations/Compare To Zero  relop=>  OutDataTypeStr=boolean
  Demux : Demux  Outputs=3
  Gain : Gain  Gain=motor.p
  Mux : Mux  Inputs=3
  Mux1 : Mux  Inputs=3
  Trigonometric Function : Trigonometry  Operator=cos
  Hall : Outport
  wires:
  Bias1/1 -> Mux/2
  Angle/1 -> Gain/1
  Trigonometric Function/1 -> Demux/1
  Compare To Zero1/1 -> Mux1/2  "H2"
  Bias/1 -> Mux/1
  Mux1/1 -> Hall/1
  Gain/1 -> Bias2/1, Bias1/1, Bias/1
  Compare To Zero2/1 -> Mux1/3  "H3"
  Demux/3 -> Compare To Zero2/1
  Bias2/1 -> Mux/3
  Mux/1 -> Trigonometric Function/1
  Demux/2 -> Compare To Zero1/1
  Compare To Zero3/1 -> Mux1/1  "H1"
  Demux/1 -> Compare To Zero3/1

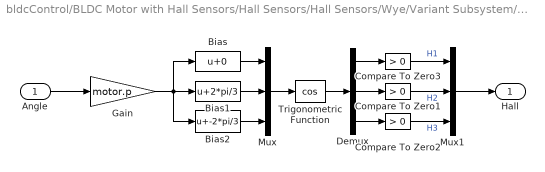
== system bldcControl/BLDC Motor with Hall Sensors/Hall Sensors/Hall Sensors/Wye/Variant Subsystem/120 degree ==
  Angle : Inport
  Bias : Bias
  Bias1 : Bias  Bias=2*pi/3
  Bias2 : Bias  Bias=-2*pi/3
  Compare To Zero1 : simulink/Logic and Bit Operations/Compare To Zero  relop=>  OutDataTypeStr=boolean
  Compare To Zero2 : simulink/Logic and Bit Operations/Compare To Zero  relop=>  OutDataTypeStr=boolean
  Compare To Zero3 : simulink/Logic and Bit Operations/Compare To Zero  relop=>  OutDataTypeStr=boolean
  Demux : Demux  Outputs=3
  Gain : Gain  Gain=motor.p
  Mux : Mux  Inputs=3
  Mux1 : Mux  Inputs=3
  Trigonometric Function : Trigonometry  Operator=cos
  Hall : Outport
  wires:
  Bias2/1 -> Mux/3
  Mux1/1 -> Hall/1
  Demux/3 -> Compare To Zero2/1
  Mux/1 -> Trigonometric Function/1
  Gain/1 -> Bias/1, Bias2/1, Bias1/1
  Compare To Zero1/1 -> Mux1/2  "H2"
  Compare To Zero3/1 -> Mux1/1  "H1"
  Trigonometric Function/1 -> Demux/1
  Bias1/1 -> Mux/2
  Bias/1 -> Mux/1
  Compare To Zero2/1 -> Mux1/3  "H3"
  Demux/2 -> Compare To Zero1/1
  Demux/1 -> Compare To Zero3/1
  Angle/1 -> Gain/1

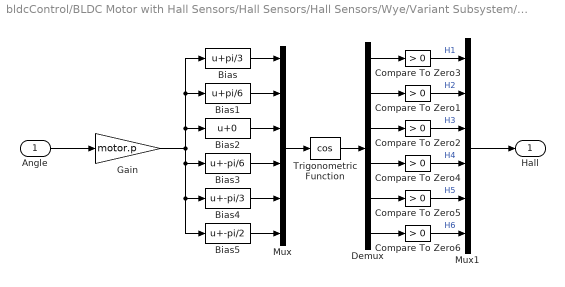
== system bldcControl/BLDC Motor with Hall Sensors/Hall Sensors/Hall Sensors/Wye/Variant Subsystem/150 degree ==
  Angle : Inport
  Bias : Bias  Bias=pi/3
  Bias1 : Bias  Bias=pi/6
  Bias2 : Bias
  Bias3 : Bias  Bias=-pi/6
  Bias4 : Bias  Bias=-pi/3
  Bias5 : Bias  Bias=-pi/2
  Compare To Zero{1..6} (6 alike) : simulink/Logic and Bit Operations/Compare To Zero  relop=>  OutDataTypeStr=boolean
  Demux : Demux  Outputs=6
  Gain : Gain  Gain=motor.p
  Mux : Mux  Inputs=6
  Mux1 : Mux  Inputs=6
  Trigonometric Function : Trigonometry  Operator=cos
  Hall : Outport
  wires:
  Bias5/1 -> Mux/6
  Compare To Zero6/1 -> Mux1/6  "H6"
  Bias4/1 -> Mux/5
  Bias3/1 -> Mux/4
  Mux1/1 -> Hall/1
  Bias2/1 -> Mux/3
  Bias1/1 -> Mux/2
  Demux/1 -> Compare To Zero3/1
  Compare To Zero4/1 -> Mux1/4  "H4"
  Demux/6 -> Compare To Zero6/1
  Bias/1 -> Mux/1
  Demux/5 -> Compare To Zero5/1
  Mux/1 -> Trigonometric Function/1
  Compare To Zero5/1 -> Mux1/5  "H5"
  Demux/4 -> Compare To Zero4/1
  Compare To Zero3/1 -> Mux1/1  "H1"
  Angle/1 -> Gain/1
  Trigonometric Function/1 -> Demux/1
  Demux/2 -> Compare To Zero1/1
  Gain/1 -> Bias2/1, Bias1/1, Bias/1, Bias5/1, Bias4/1, Bias3/1
  Demux/3 -> Compare To Zero2/1
  Compare To Zero1/1 -> Mux1/2  "H2"
  Compare To Zero2/1 -> Mux1/3  "H3"

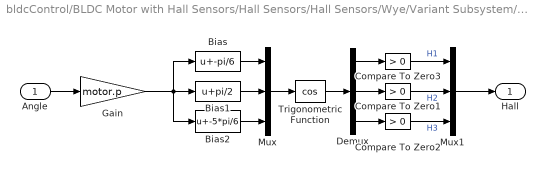
== system bldcControl/BLDC Motor with Hall Sensors/Hall Sensors/Hall Sensors/Wye/Variant Subsystem/180 degree ==
  Angle : Inport
  Bias : Bias  Bias=-pi/6
  Bias1 : Bias  Bias=pi/2
  Bias2 : Bias  Bias=-5*pi/6
  Compare To Zero1 : simulink/Logic and Bit Operations/Compare To Zero  relop=>  OutDataTypeStr=boolean
  Compare To Zero2 : simulink/Logic and Bit Operations/Compare To Zero  relop=>  OutDataTypeStr=boolean
  Compare To Zero3 : simulink/Logic and Bit Operations/Compare To Zero  relop=>  OutDataTypeStr=boolean
  Demux : Demux  Outputs=3
  Gain : Gain  Gain=motor.p
  Mux : Mux  Inputs=3
  Mux1 : Mux  Inputs=3
  Trigonometric Function : Trigonometry  Operator=cos
  Hall : Outport
  wires:
  Bias1/1 -> Mux/2
  Angle/1 -> Gain/1
  Trigonometric Function/1 -> Demux/1
  Compare To Zero1/1 -> Mux1/2  "H2"
  Bias/1 -> Mux/1
  Mux1/1 -> Hall/1
  Gain/1 -> Bias1/1, Bias2/1, Bias/1
  Compare To Zero2/1 -> Mux1/3  "H3"
  Demux/3 -> Compare To Zero2/1
  Bias2/1 -> Mux/3
  Mux/1 -> Trigonometric Function/1
  Demux/2 -> Compare To Zero1/1
  Compare To Zero3/1 -> Mux1/1  "H1"
  Demux/1 -> Compare To Zero3/1
